simulink model "dpsim_rlc_3ph_reference"  (R2025a)
settings: Solver=ode45  StartTime=0  StopTime=0.10000000000000001  MaxStep=1.0000000000000001e-05  RelTol=1e-9  AbsTol=1e-10
settings Model: Creator=matthiasmees  LastModifiedBy=matthiasmees

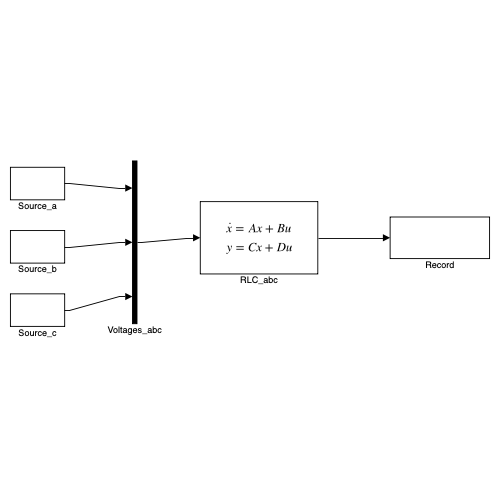
[thumbnail: Simulink's stored preview of the top-level diagram]
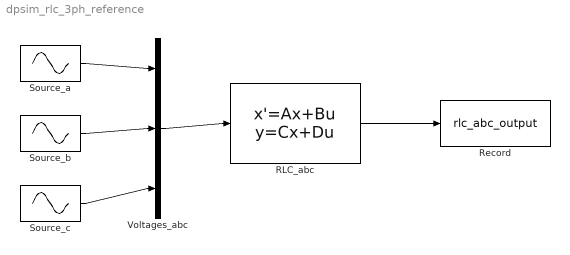
== system dpsim_rlc_3ph_reference ==
  RLC_abc : StateSpace  A=[-500 0 0 -50 0 0;0 -500 0 0 -50 0;0 0 -500 0 0 -50;10000 0 0 0 0 0;0 10000 0 0 0 0;0 0 10000 0 0 0]  B=[50 0 0;0 50 0;0 0 50;0 0 0;0 0 0;0 0 0]  C=[1 0 0 0 0 0;0 1 0 0 0 0;0 0 1 0 0 0;0 0 0 1 0 0;0 0 0 0 1 0;0 0 0 0 0 1]  D=[0 0 0;0 0 0;0 0 0;0 0 0;0 0 0;0 0 0]  InitialCondition=[0;0;0;0;0;0]
  Record : ToWorkspace  VariableName=rlc_abc_output  SaveFormat=Timeseries  SampleTime=-1
  Source_a : Sin  Amplitude=325.26911934581187  Frequency=314.15926535897933  SampleTime=0
  Source_b : Sin  Amplitude=325.26911934581187  Frequency=314.15926535897933  Phase=-2.0943951023931953  SampleTime=0
  Source_c : Sin  Amplitude=325.26911934581187  Frequency=314.15926535897933  Phase=2.0943951023931953  SampleTime=0
  Voltages_abc : Mux  Inputs=3
  wires:
  Source_a/1 -> Voltages_abc/1
  Source_b/1 -> Voltages_abc/2
  Source_c/1 -> Voltages_abc/3
  Voltages_abc/1 -> RLC_abc/1
  RLC_abc/1 -> Record/1
